simulink model "EXPT2_without_bypass"  (R2024a)
settings: Solver=VariableStepAuto  StartTime=0.0  StopTime=1  RelTol=1e-3
undefined symbols (not defined in the file): powergui, sps_lib
libraries: spsPVArrayLib x2, spsControlledVoltageSourceLib x1, spsCurrentMeasurementLib x1, spsDiodeLib x1, simulink x1, spsVoltageMeasurementLib x1
settings Model: Creator=A Harish  LastModifiedBy=Aswin
settings OptimizationCC: ReuseModelBlockBuffer=off
settings RTWCC: GPUComputeCapability=3.5

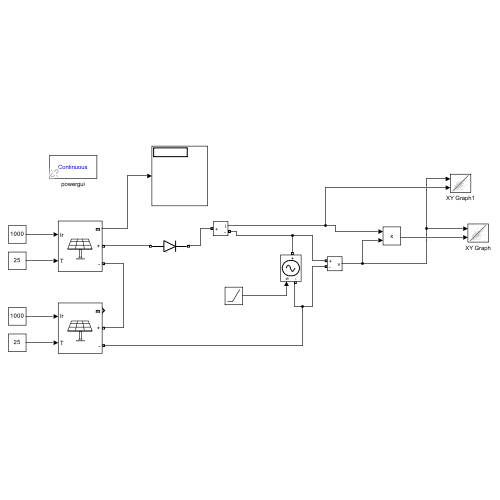
[thumbnail: Simulink's stored preview of the top-level diagram]
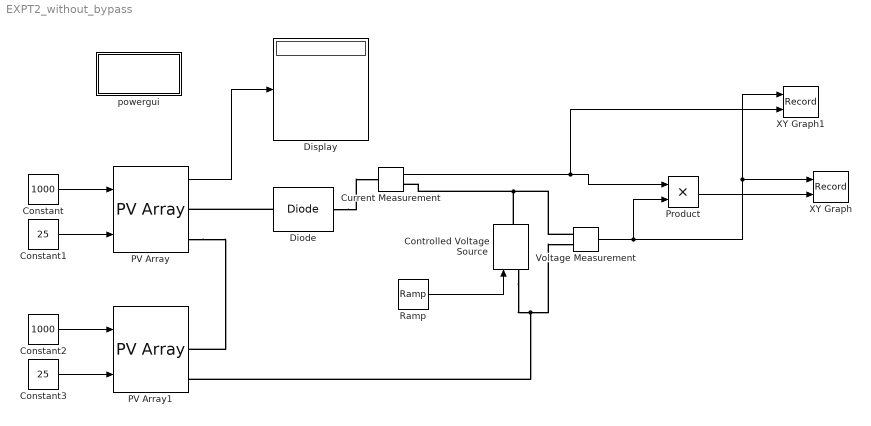
== system EXPT2_without_bypass ==
  Constant : Constant  Value=1000
  Constant1 : Constant  Value=25
  Constant2 : Constant  Value=1000
  Constant3 : Constant  Value=25
  Controlled Voltage Source : spsControlledVoltageSourceLib/Controlled Voltage Source  Initialize=on  Source_Type=DC  Amplitude=0  Phase=0  Frequency=0  Measurements=None
  Current Measurement : spsCurrentMeasurementLib/Current Measurement  PhasorSimulation=off  OutputType=Complex  PSBequivalent=0
  Diode : spsDiodeLib/Diode  Ron=0.001  Lon=0  Vf=0.8  IC=0  UseSnubber=0  Rs=0  Cs=0  Measurements=off
  Display : Display
  PV Array : spsPVArrayLib/PV Array  Npar=1  Nser=1  PlotType=array @ 1000 W/m2 & specified temperatures  S_vec="[ 1000  500  100 ]"  Temp_C_vec="[ 45 25  ]"  ModuleName=User-defined  PlotWhenSelected=off  Pm=166.9842  Ncell=36  Voc=22.5  Isc=9.11  Vm=19.26  Im=8.67  beta_Voc_pc=-0.36099  alpha_Isc_pc=0.102  beta_Voc=-0.081223  alpha_Isc=0.0092922  IL=9.1344  I0=3.4087e-10  nI=1.0133  Rsh=462.5172  Rs=0.043489  RobustModel=off  RobustCellTemperature=313.3991  BAL=on  Tc=1e-6  Tfilter=5e-5
  PV Array1 : spsPVArrayLib/PV Array  Npar=1  Nser=1  PlotType=array @ 1000 W/m2 & specified temperatures  S_vec="[ 1000  500  100 ]"  Temp_C_vec="[ 45 25  ]"  ModuleName=User-defined  PlotWhenSelected=off  Pm=166.9842  Ncell=36  Voc=22.5  Isc=9.11  Vm=19.26  Im=8.67  beta_Voc_pc=-0.36099  alpha_Isc_pc=0.102  beta_Voc=-0.081223  alpha_Isc=0.0092922  IL=9.1344  I0=3.4087e-10  nI=1.0133  Rsh=462.5172  Rs=0.043489  RobustModel=off  RobustCellTemperature=313.3991  BAL=on  Tc=1e-6  Tfilter=5e-5
  Product : Product
  Ramp : simulink/Sources/Ramp  slope=2.25  start=0  InitialOutput=0
  Voltage Measurement : spsVoltageMeasurementLib/Voltage Measurement  PhasorSimulation=off  OutputType=Complex  PSBequivalent=0
  XY Graph : Record  FileSettingsInternal="{\"entries\":[{\"content\":{\"excelSettings\":{\"content\":{},\"type\":\"Streamout.ExcelSettings\"}},\"type\":\"Streamout.FileSettingStorage\",\"uuid\":\"\"}],\"packageUris\":[\"http:\\/\\/schema.mathworks.com\\/mf0\\/streamout_blocks\\/R2020a\"],\"version\":\"1.0\"}"  Layout=[1 1]  SignalsInternal="{\"entries\":[{\"content\":{\"signals\":[{\"content\":{\"blockPath\":[],\"dimensions\":[1],\"domain\":\"\",\"lineColor\":\"#a2142f\",\"plots\":[ 1 ],\"port\":1,\"signalID\":1,\"signalName\":\"Voltage Measurement\"},\"type\":\"RecordBlkView.Signal\",\"uuid\":\"\"},{\"content\":{\"blockPath\":[],\"dimensions\":[1],\"domain\":\"\",\"lineColor\":\"#139fff\",\"plots\":[ 1 ],\"port\":2,\"signalID\":2,\"signalName\":\"Product\"},\"type\":\"RecordBlkView.Signal\",\"uuid\":\"\"}]},\"type\":\"RecordBlkView.InputSignals\",\"uuid\":\"\"}],\"packageUris\":[\"http:\\/\\/schema.mathworks.com\\/mf0\\/streamout_blocks\\/R2020a\"],\"version\":\"1.0\"}"  VisualizationBindings="{\"xyplotplugin\":{\"info\":[{\"series\":[{\"bindingParametersList\":[{\"parameter\":\"X-Axis\",\"signalID\":1,\"signalName\":\"Voltage Measurement\"},{\"parameter\":\"Y-Axis\",\"signalID\":2,\"signalName\":\"Product\"}],\"seriesID\":0}],\"subplotID\":1}]}}"  CompatibilityTag=XY
  XY Graph1 : Record  FileSettingsInternal="{\"entries\":[{\"content\":{\"excelSettings\":{\"content\":{},\"type\":\"Streamout.ExcelSettings\"}},\"type\":\"Streamout.FileSettingStorage\",\"uuid\":\"\"}],\"packageUris\":[\"http:\\/\\/schema.mathworks.com\\/mf0\\/streamout_blocks\\/R2020a\"],\"version\":\"1.0\"}"  Layout=[1 1]  SignalsInternal="{\"entries\":[{\"content\":{\"signals\":[{\"content\":{\"blockPath\":[],\"dimensions\":[1],\"domain\":\"\",\"lineColor\":\"#a2142f\",\"plots\":[ 1 ],\"port\":1,\"signalID\":1,\"signalName\":\"Voltage Measurement\"},\"type\":\"RecordBlkView.Signal\",\"uuid\":\"\"},{\"content\":{\"blockPath\":[],\"dimensions\":[1],\"domain\":\"\",\"lineColor\":\"#139fff\",\"plots\":[ 1 ],\"port\":2,\"signalID\":2,\"signalName\":\"Current Measurement\"},\"type\":\"RecordBlkView.Signal\",\"uuid\":\"\"}]},\"type\":\"RecordBlkView.InputSignals\",\"uuid\":\"\"}],\"packageUris\":[\"http:\\/\\/schema.mathworks.com\\/mf0\\/streamout_blocks\\/R2020a\"],\"version\":\"1.0\"}"  VisualizationBindings="{\"xyplotplugin\":{\"info\":[{\"series\":[{\"bindingParametersList\":[{\"parameter\":\"X-Axis\",\"signalID\":1,\"signalName\":\"Voltage Measurement\"},{\"parameter\":\"Y-Axis\",\"signalID\":2,\"signalName\":\"Current Measurement\"}],\"seriesID\":0}],\"subplotID\":1}]}}"  CompatibilityTag=XY
  powergui : Subsystem  Priority=1  AncestorBlock=sps_lib/powergui  InitFcn=powergui( 'InitFcn_Callback' , gcb , 0 , [ ] );  mask(PSB option menu block){SimulationMode=Continuous, SampleTime=50e-6, frequency=60, Iterations=50, frequencyindice=0, Pbase=100e6, ErrMax=1e-4, UnitsV=kV, UnitsW=MW, buscounter=0, FunctionMessages=off, echomessages=off, EnableUseOfTLC=off, CurrentSourceSwitches=off, DisableSnubberDevices=off, DisableRonSwitches=off, DisableVfSwitches=off, DisplayEquations=off, AutomaticDiscreteSolvers=off, SolverType=Tustin/Backward Euler (TBE), Interpol=off, ExternalGateDelay=off, methode=off, Ts=100, x0status=blocks, SPID=on, SwTol=0, HookPort=off, NonlinearTolerance=1e-4, nMaxIteration=100, ContinueOnMaxIteration=off, RestoreLinks=warning, ResistiveCurrentMeasurement=off, Frange=[0:2:500], Ylog=off, Xlog=on, ShowGrid=off, save=off, variable=ZData, structure=0, ZoomFFT=off, StartTime=0.0, cycles=1, DisplayStyle=1, fundamental=60, FreqAxis=off, MaxFrequency=1000, frequencyindicesteady=1, RmsSteady=1, display=off}
      mask prompts: SimulationMode "Simulation type:"; SampleTime "Sample time (s):"; frequency "Frequency (Hz):"; Iterations "Max iterations"; frequencyindice "Frequency (Hz)"; Pbase "Base power (VA)"; ErrMax "PQ tolerance (pu)"; UnitsV "Voltage units"; UnitsW "Power units"; buscounter "Load flow bus counter"; FunctionMessages "Disable Specialized Power Systems warnings"; echomessages "Display Specialized Power Systems compilation messages"; EnableUseOfTLC "Use TLC file when in Accelerator Simulation Mode and for code generation"; CurrentSourceSwitches "Disable ideal switching"; DisableSnubberDevices "Disable snubbers in switching devices"; DisableRonSwitches "Disable Ron resistances in switching devices"; DisableVfSwitches "Disable forward voltages in switching devices"; DisplayEquations "Display circuit differential equations"; AutomaticDiscreteSolvers "Automatically handle Discrete solver and Advanced tab solver settings of blocks"; SolverType "Discrete solver"; Interpol "Interpolate switching events"; ExternalGateDelay "Use time-stamped gate signals"; methode "Store switching topologies"; Ts "Buffer size (MBytes):"; x0status "Start simulation with initial electrical states from:"; SPID "Use ideal switching devices"; SwTol "Switch tolerance"; HookPort "Allow multiple powergui blocks"; NonlinearTolerance "Solver tolerance"; nMaxIteration "Maximum number of iterations"; ContinueOnMaxIteration "Continue Simulation if maximum number of iterations is reached"; RestoreLinks "Restore disabled links of Simscape Power Systems ST blocks:"; ResistiveCurrentMeasurement "Use non ideal current measurement blocks (1e-4Ohm internal resistance)"; Frange "Frequency Range"; Ylog "Log impedance"; Xlog "log Frequency"; ShowGrid "grid"; save "Save Data To Workspace"; variable "Variable Name"; structure "Structure Name (PSBFFTSCOPE)"; ZoomFFT "ZoomFFT (PSBFFTSCOPE)"; StartTime "Start Time (PSBFFTSCOPE)"; cycles "Cycles (PSBFFTSCOPE)"; DisplayStyle "Display style (PSBFFTSCOPE)"; fundamental "Fundamental (PSBFFTSCOPE)"; FreqAxis "Frequency Axis (PSBFFTSCOPE)"; MaxFrequency "Max Frequency (PSBFFTSCOPE)"; frequencyindicesteady "Frequency indice (STEADYSTATE)"; RmsSteady "RMS display (STEADYSTATE)"; display "Display Results"
      mask help: Set simulation type, simulation parameters, and preferences.
      mask init:
      | dispMessage = '';
      | dispMessage = powergui('MaskInitialization',gcb,SimulationMode,SampleTime);
      settings: LibrarySourceBlock=sps_lib/powergui  PreSaveFcn=powergui( 'PreSaveFcn_Callback' , gcb , [ ] , [ ] );  OpenFcn=sps_rtmsupport('OpenFcn',gcbh)
      mask Help: helpview(psbhelp)
      mask TypeOptions SimulationMode: Continuous | Discrete | Phasor | Discrete phasor
      mask Callback SimulationMode: powergui('SimulationType',[],[],gcb);
      mask TypeOptions UnitsV: V | kV
      mask TypeOptions UnitsW: W | kW | MW
      mask Callback CurrentSourceSwitches: powergui('SimulationType',[],[],gcb);
      mask Callback AutomaticDiscreteSolvers: powergui('SimulationType',[],[],gcb);
      mask TypeOptions SolverType: Tustin/Backward Euler (TBE) | Tustin | Backward Euler
      mask Callback SolverType: powergui('SimulationType',[],[],gcb);
      mask Callback Interpol: powergui('SimulationType',[],[],gcb);
      mask Callback ExternalGateDelay: powergui('SimulationType',[],[],gcb);
      mask Callback methode: powergui('SimulationType',[],[],gcb);
      mask TypeOptions x0status: blocks | steady | zero
      mask TypeOptions RestoreLinks: yes | warning | no
      mask Callback display: sps_rtmsupport('parametereditingmodes',gcbh) % Will be executed last in parameter callbacks to ensure mask enable consistency
      mask DialogControl SolverTab Prompt: Solver
      mask DialogControl AutoSolverNote Prompt: The Simulation type parameter is governed by Simulink. To access the Powergui solver settings, unselect auto (Automatic solver selection) solver in the Simulink solver options.
      mask DialogControl Apps Prompt: Apps
      mask DialogControl StateAnalyzer Prompt: Measurements and States Analyzer
      mask DialogControl StateAnalyzer Callback: powerStates(bdroot(gcb))
      mask DialogControl LineParameterCalculator Prompt: Line Parameter Calculator
      mask DialogControl LineParameterCalculator Callback:
      | close_system(gcb)
      | powerLineParameters
      mask DialogControl CableParameterCalculator Prompt: Cable Parameter Calculator
      mask DialogControl CableParameterCalculator Callback:
      | close_system(gcb)
      | powerCableParameters
      mask DialogControl LineDecoupler Prompt: Line Decoupler
      mask DialogControl LineDecoupler Tooltip: Click to replace selected Distributed Parameters Line blocks with Decoupling Line blocks
      mask DialogControl LineDecoupler Callback:
      | close_system(gcb);
      | DecouplingLineReplace(gcs)
      mask DialogControl LoadFlowAnalyzer Prompt: Load Flow Analyzer
      mask DialogControl LoadFlowAnalyzer Callback:
      | close_system(gcb)
      | powerLoadFlow
      mask DialogControl LoadFlowParameters Prompt: Load Flow Parameters
      mask DialogControl ImpedanceCalculator Prompt: Impedance Calculator
      mask DialogControl ImpedanceCalculator Callback:
      | close_system(gcb);
      | powerImpedance(bdroot(gcs));
      mask DialogControl FFTAnalyzer Prompt: FFT Analyzer
      mask DialogControl FFTAnalyzer Callback:
      | close_system(gcb)
      | power_fftscope(bdroot(gcb),gcb)
      mask DialogControl LinearSystemAnalyzer Prompt: Linear System Analyzer
      mask DialogControl LinearSystemAnalyzer Callback:
      | close_system(gcb)
      | power_ltiview(bdroot(gcb))
      mask DialogControl HysteresisDesigner Prompt: Hysteresis Designer
      mask DialogControl HysteresisDesigner Callback:
      | close_system(gcb)
      | powerHysteresis('hysteresis.mat')
      mask DialogControl BlockCustomizer Prompt: Block Customizer
      mask DialogControl BlockCustomizer Callback:
      | close_system(gcb);
      | power_customize;
      mask DialogControl ReportGenerator Prompt: Report Generator
      mask DialogControl ReportGenerator Callback:
      | close_system(gcb)
      | power_report(bdroot(gcb))
      mask DialogControl obsolete Prompt: ...
      mask DialogControl MachineInitialization Prompt: Machine Initialization
      mask DialogControl MachineInitialization Callback:
      | close_system(gcb)
      | powericon('machineInitTool',bdroot(gcb),gcb)
      mask DialogControl Preferences Prompt: Preferences
      mask DialogControl Solver Prompt: Solver
      mask DialogControl SolverDetails Prompt: Solver details for nonlinear elements
      mask Display: color('blue'),disp(dispMessage)
  wires:
  PV Array/1 -> Display/1
  Constant/1 -> PV Array/1
  Constant1/1 -> PV Array/2
  Ramp/1 -> Controlled Voltage Source/1
  Current Measurement/1 -> XY Graph1/2, Product/1
  Voltage Measurement/1 -> Product/2, XY Graph1/1, XY Graph/1
  Product/1 -> XY Graph/2
  Constant3/1 -> PV Array1/2
  Constant2/1 -> PV Array1/1
  connections:
  Controlled Voltage Source/RConn1 -- Current Measurement/RConn1 -- Voltage Measurement/LConn1
  Diode/LConn1 -- PV Array/RConn1
  Diode/RConn1 -- Current Measurement/LConn1
  PV Array/RConn2 -- PV Array1/RConn1
  Controlled Voltage Source/LConn1 -- PV Array1/RConn2 -- Voltage Measurement/LConn2

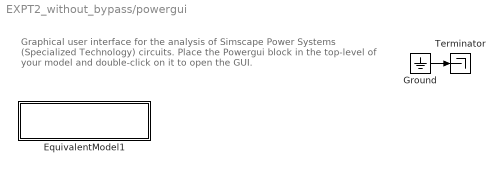
== system EXPT2_without_bypass/powergui ==
  note: Graphical user interface for the analysis of
      | Simscape Power Systems (Specialized Technology) circuits.
      | Place the Powergui block in the top-level of your model and double-click
      | on it to open the GUI.
  EquivalentModel1 : Subsystem  mask{SwTol=SwTol}
      mask prompts: SwTol "SwitchTolerance"
      mask init:
      | S  = GetDataForEquivalentModel('SPID',gcbh,SwTol);
      mask Display:
      | color('blue')
      | disp('EQUIVALENT CIRCUIT\nSPID')
  Ground : Ground
  Terminator : Terminator
  wires:
  Ground/1 -> Terminator/1

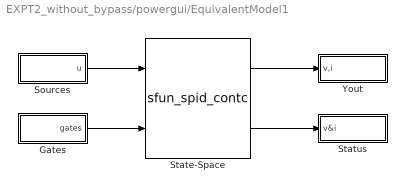
== system EXPT2_without_bypass/powergui/EquivalentModel1 ==
  Gates : Subsystem
  Sources : Subsystem
  State-Space : S-Function  FunctionName=sfun_spid_contc  Parameters=S.Mg, [S.nb.x S.nb.u S.nb.y S.nb.s], S.x0, S.MgColNames, S.SwitchVf, S.SwitchType, S.SwitchGateInitialValue, S.SwitchTolerance,S.SaveMatrices,S.BufferSize  SFunctionDeploymentMode=off  EnableBusSupport=off
  Status : Subsystem
  Yout : Subsystem
  wires:
  State-Space/1 -> Yout/1(v,i)
  State-Space/2 -> Status/1(v&i)
  Gates/1(gates) -> State-Space/2
  Sources/1(u) -> State-Space/1

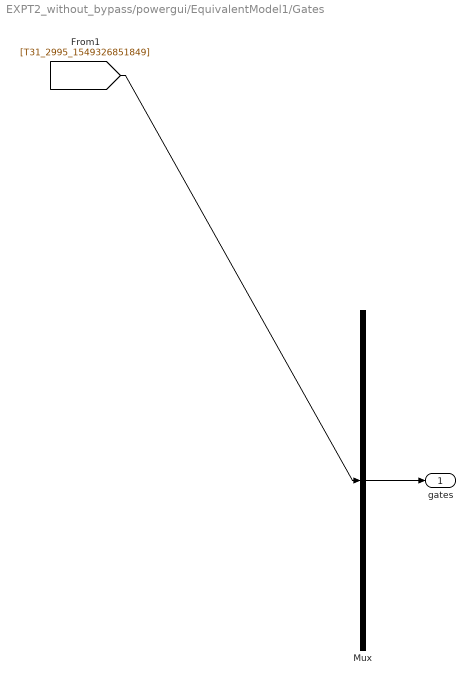
== system EXPT2_without_bypass/powergui/EquivalentModel1/Gates ==
  Mux : Mux  Inputs=1
  gates : Outport  VectorParamsAs1DForOutWhenUnconnected=off
  wires:
  Mux/1 -> gates/1
  [T31_2995_1549326851849] -> Mux/1

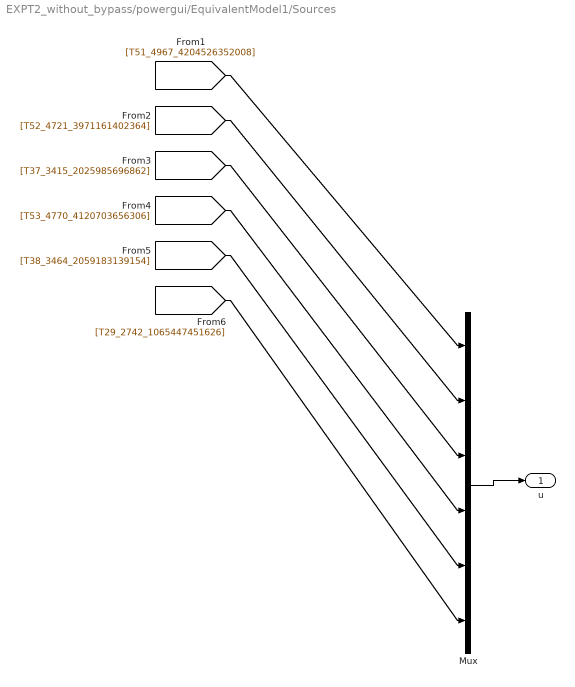
== system EXPT2_without_bypass/powergui/EquivalentModel1/Sources ==
  Mux : Mux  Inputs=[1 1 1 1 1 1]
  u : Outport  VectorParamsAs1DForOutWhenUnconnected=off
  wires:
  Mux/1 -> u/1
  [T51_4967_4204526352008] -> Mux/1
  [T52_4721_3971161402364] -> Mux/2
  [T37_3415_2025985696862] -> Mux/3
  [T53_4770_4120703656306] -> Mux/4
  [T38_3464_2059183139154] -> Mux/5
  [T29_2742_1065447451626] -> Mux/6

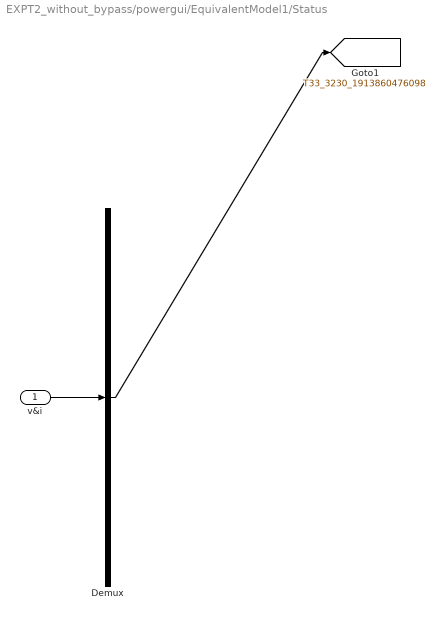
== system EXPT2_without_bypass/powergui/EquivalentModel1/Status ==
  v&i : Inport
  Demux : Demux  Outputs=1
  tag scope: T33_3230_1913860476098=global
  wires:
  v&i/1 -> Demux/1
  Demux/1 -> [T33_3230_1913860476098]

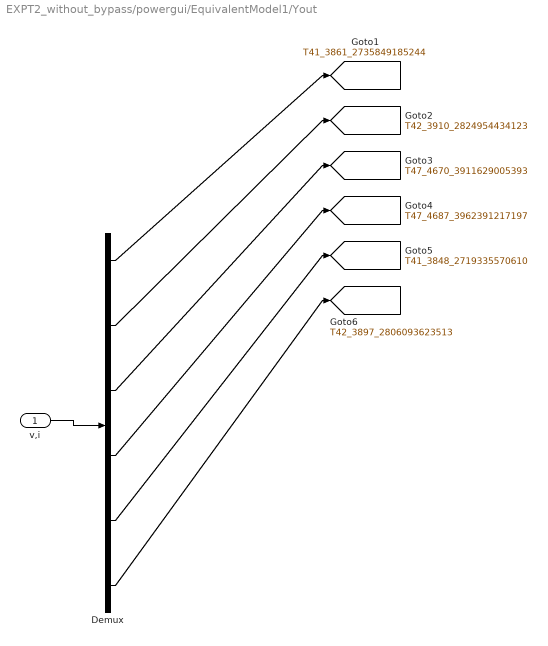
== system EXPT2_without_bypass/powergui/EquivalentModel1/Yout ==
  v,i : Inport
  Demux : Demux  Outputs=[1 1 1 1 1 1]
  tag scope: T41_3848_2719335570610=global, T41_3861_2735849185244=global, T42_3897_2806093623513=global, T42_3910_2824954434123=global, T47_4670_3911629005393=global, T47_4687_3962391217197=global
  wires:
  v,i/1 -> Demux/1
  Demux/1 -> [T41_3861_2735849185244]
  Demux/2 -> [T42_3910_2824954434123]
  Demux/3 -> [T47_4670_3911629005393]
  Demux/4 -> [T47_4687_3962391217197]
  Demux/5 -> [T41_3848_2719335570610]
  Demux/6 -> [T42_3897_2806093623513]
